simulink model "gtm_design_lpv"  (R2021b)
settings: Solver=VariableStepAuto  StartTime=0.0  StopTime=10  FixedStep=0.005  MaxStep=0.005  RelTol=1e-3
StopFcn:
  | MWSout=grabmws(bdroot);
  | MWSout.lastrun=datestr(now);
values from neighbouring files (symbols this model uses):
  s = tf('s')    [SingleDOF.m]    (also in main.m; mainSimple.m; newmain.m)
undefined symbols (not defined in the file or in its folder): Aero, aftfuel, aftfuel_pos, AILL, AILLC, AILR, AILRC, alpha_deg, altitude_ft, Ax_g, Ay_g, Az_g, b, beta_deg, bias, BRAKEC, Cbar, cg_pos0, cg_shift_gear, DamageCase, DamageModels, DamageOnsetTime, Earth, ELLIB, ELLIBC, ELLOB, ELLOBC, ELRIB, ELRIBC, ELROB, ELROBC, engl_ang, engl_pos, engr_ang, engr_pos, FLAPLIB, FLAPLIC, FLAPLOB, FLAPLOC, FLAPRIB, FLAPRIC, FLAPROB, FLAPROC, ft, FuelUsed_Init, fwdfuel, fwdfuel_pos, GEAR, GEARC, Inertia0, Inertia_shift_gear, Ixx_model, Iyy_model, Izz_model, KTAS, LandingGear, LengON, LinearizeModeOn, NAV_altitude_m, NAV_latitude_deg ... (+51)
libraries: simulink_extras x63, simulink_need_slupdate x30, LPVBlockLibrary x20, aerolibconvert2 x6, aerolibtransform2 x5, uavalgslib x4, UserContent_lib x3, simulink x3, robotcorelib x1, uavutilslib x1
(part 5 of 8)

== system gtm_design_lpv/GTM_T2/Sensors/MIDG II 50 Hz ==
  AuxVars : Inport
  EOM_State : Inport  Port=2
  0.01 deg Resolution : Quantizer  QuantizationInterval=0.01
  0.01 deg Resolution1 : Quantizer  QuantizationInterval=0.01
  0.01 deg Resolution2 : Quantizer  QuantizationInterval=0.01
  0.01 m Resolution1 : Quantizer  QuantizationInterval=0.01
  0.01 m/s Resolution : Quantizer  QuantizationInterval=0.01
  0.01 m/s Resolution1 : Quantizer  QuantizationInterval=0.01
  0.01 m/s Resolution2 : Quantizer  QuantizationInterval=0.01
  1e-7 deg Resolution2 : Quantizer  QuantizationInterval=1e-7
  1e-7 deg Resolution3 : Quantizer  QuantizationInterval=1e-7
  Bus Selector3 : BusSelector  OutputSignals=phi,theta,psi,latitude,longitude,altitude
  Bus Selector8 : BusSelector  OutputSignals=Vn,Ve,Vd
  Bus to Vector : BusToVector
  Gain10 : Gain  Gain=0.5144
  Gain11 : Gain  Gain=-0.5144
  Gain12 : Gain  Gain=0.3048
  Gain{13..17} (5 alike) : Gain  Gain=180/pi
  Gain9 : Gain  Gain=0.5144
  MIDG Labels : Subsystem
  MIDG bus : BusCreator  Inputs=9
  Map+/-180 : Subsystem
  Rate Transition : RateTransition
  Scope{,1..4} (5 alike) : Scope
  Selector{,1..3} (4 alike) : Selector  InputPortWidth=9  IndexOptions=Index vector (dialog)  Indices=4  OutputSizes=1
  Sensor Model7 : Subsystem  mask(Sensor Model){noise_on=SensorNoise.On, sigma=SensorNoise.MIDG.psi.Std, seed=878232, bias=SensorNoise.MIDG.psi.Bias, scf=SensorNoise.MIDG.psi.Scf}
      mask prompts: noise_on "on/off"; scf "scale factor:"
      mask help:
      | Add bias, scale factor, and white noise to a signal
      |
      | - 'on/off': 1 = noise on, 0 = noise off.
      | - 'sigma' : Standard deviation of white noise.
      | - 'seed'  : Random number seed. Generated numbers
      |   change between each simulation run, but the random number
      |   sequences do not change between Matlab sessions unless a
      |   new seed is specified.
      | - 'bias'  : Constant mean value offset of white noise.
      | - 'scale factor' : Scale factor applied to original signal.
      mask Display: disp('bias/scf/noise')
  Sensor Model8 : Subsystem  mask(Sensor Model){noise_on=SensorNoise.On, sigma=SensorNoise.MIDG.theta.Std, seed=878231, bias=SensorNoise.MIDG.theta.Bias, scf=SensorNoise.MIDG.theta.Scf}
      mask prompts: noise_on "on/off"; scf "scale factor:"
      mask help:
      | Add bias, scale factor, and white noise to a signal
      |
      | - 'on/off': 1 = noise on, 0 = noise off.
      | - 'sigma' : Standard deviation of white noise.
      | - 'seed'  : Random number seed. Generated numbers
      |   change between each simulation run, but the random number
      |   sequences do not change between Matlab sessions unless a
      |   new seed is specified.
      | - 'bias'  : Constant mean value offset of white noise.
      | - 'scale factor' : Scale factor applied to original signal.
      mask Display: disp('bias/scf/noise')
  Sensor Model9 : Subsystem  mask(Sensor Model){noise_on=SensorNoise.On, sigma=SensorNoise.MIDG.phi.Std, seed=878230, bias=SensorNoise.MIDG.phi.Bias, scf=SensorNoise.MIDG.phi.Scf}
      mask prompts: noise_on "on/off"; scf "scale factor:"
      mask help:
      | Add bias, scale factor, and white noise to a signal
      |
      | - 'on/off': 1 = noise on, 0 = noise off.
      | - 'sigma' : Standard deviation of white noise.
      | - 'seed'  : Random number seed. Generated numbers
      |   change between each simulation run, but the random number
      |   sequences do not change between Matlab sessions unless a
      |   new seed is specified.
      | - 'bias'  : Constant mean value offset of white noise.
      | - 'scale factor' : Scale factor applied to original signal.
      mask Display: disp('bias/scf/noise')
  TimeDelay with IC feedthrough : Subsystem  mask{TimeDelay=40e-3}
      mask prompts: TimeDelay "Time Delay (sec)"
      mask help:
      | Implements Continuous Time Transport Delay with initial
      | outputs set to feedthrough with no delay.
      |
      |   output = input;   for t<TimeDelay
      |   output = input(t-tdelay); for t>=TimeDelay
  Zero-Order Hold : ZeroOrderHold  SampleTime=round(1/Timestep/50)*Timestep
  MIDG : Outport
  wires:
  Bus to Vector/1 -> Selector/1, TimeDelay with IC feedthrough/1(I)
  TimeDelay with IC feedthrough/1(O) -> Selector1/1, Zero-Order Hold/1
  MIDG bus/1 -> Bus to Vector/1
  Zero-Order Hold/1 -> Selector2/1, Rate Transition/1
  EOM_State/1 -> Bus Selector3/1
  Bus Selector3/1 -> Gain13/1  "<phi>"
  Bus Selector3/2 -> Gain14/1  "<theta>"
  Bus Selector3/3 -> Gain15/1  "<psi>"
  Sensor Model7/1(Out1) -> 0.01 deg Resolution2/1
  Sensor Model8/1(Out1) -> 0.01 deg Resolution1/1
  Sensor Model9/1(Out1) -> 0.01 deg Resolution/1
  0.01 deg Resolution/1 -> MIDG bus/1  "phi"
  0.01 deg Resolution1/1 -> MIDG bus/2  "theta"
  0.01 deg Resolution2/1 -> Map+/-180/1(I)  "psi"
  1e-7 deg Resolution2/1 -> Scope/1, MIDG bus/4  "latitude"
  1e-7 deg Resolution3/1 -> MIDG bus/5  "longitude"
  0.01 m Resolution1/1 -> MIDG bus/6  "altitude"
  Gain9/1 -> 0.01 m/s Resolution/1
  Gain10/1 -> 0.01 m/s Resolution1/1
  Gain11/1 -> 0.01 m/s Resolution2/1
  Gain12/1 -> 0.01 m Resolution1/1
  0.01 m/s Resolution/1 -> MIDG bus/7  "Vn"
  0.01 m/s Resolution1/1 -> MIDG bus/8  "Ve"
  Gain13/1 -> Sensor Model9/1(In1)
  Gain14/1 -> Sensor Model8/1(In1)
  Gain15/1 -> Sensor Model7/1(In1)
  Gain16/1 -> 1e-7 deg Resolution2/1
  Gain17/1 -> 1e-7 deg Resolution3/1
  Bus Selector8/1 -> Gain9/1  "<Vn>"
  Bus Selector8/2 -> Gain10/1  "<Ve>"
  Bus Selector8/3 -> Gain11/1  "<Vd>"
  Bus Selector3/4 -> Gain16/1  "<latitude>"
  Bus Selector3/5 -> Gain17/1  "<longitude>"
  Bus Selector3/6 -> Gain12/1  "<altitude>"
  AuxVars/1 -> Bus Selector8/1
  Map+/-180/1(O) -> MIDG bus/3  "psi"
  MIDG Labels/1(O) -> MIDG/1
  0.01 m/s Resolution2/1 -> MIDG bus/9  "Vu"
  Rate Transition/1 -> Selector3/1, MIDG Labels/1(I)
  Selector/1 -> Scope1/1
  Selector1/1 -> Scope2/1
  Selector2/1 -> Scope3/1
  Selector3/1 -> Scope4/1

== system gtm_design_lpv/GTM_T2/Sensors/Surface Pots ==
  SurfacePos : Inport
  Bus Selector : BusSelector  OutputSignals=ELLOB,ELLIB,ELROB,ELRIB,AILL,AILR,RUDU,RUDL,FLAPLIB,FLAPLOB,FLAPRIB,FLAPROB  OutputAsBus=on
  Sensor Model5 : Subsystem  mask(Sensor Model){noise_on=SensorNoise.On, sigma=SensorNoise.pots.Std, seed=878239, bias=SensorNoise.pots.Bias, scf=SensorNoise.pots.Scf}
      mask prompts: noise_on "on/off"; scf "scale factor:"
      mask help:
      | Add bias, scale factor, and white noise to a signal
      |
      | - 'on/off': 1 = noise on, 0 = noise off.
      | - 'sigma' : Standard deviation of white noise.
      | - 'seed'  : Random number seed. Generated numbers
      |   change between each simulation run, but the random number
      |   sequences do not change between Matlab sessions unless a
      |   new seed is specified.
      | - 'bias'  : Constant mean value offset of white noise.
      | - 'scale factor' : Scale factor applied to original signal.
      mask Display: disp('bias/scf/noise')
  Surface Labels : Subsystem
  Pots : Outport
  wires:
  Bus Selector/1 -> Sensor Model5/1(In1)
  SurfacePos/1 -> Bus Selector/1
  Sensor Model5/1(Out1) -> Surface Labels/1(I)
  Surface Labels/1(O) -> Pots/1

== system gtm_design_lpv/GTM_T2/TransportDelay/AntiAliasing ==
  I : Inport
  Bus Assignment : BusAssignment  AssignedSignals=AirData.alpha_deg,AirData.beta_deg,AirData.qbar_psf,AirData.KTAS,AirData.TEMPAMB_degF,AirData.altitude_ft,MAG3.p_deg,MAG3.q_deg,MAG3.r_deg,MAG3.Ax_g,MAG3.Ay_g,MAG3.Az_g,SurfacePos.ELLOB,SurfacePos.ELLIB,SurfacePos.ELROB,SurfacePos.ELRIB,SurfacePos.AILL,SurfacePos.AILR,SurfacePos.RUDU,SurfacePos.RUDL,SurfacePos.FLAPLIB,SurfacePos.FLAPLOB,SurfacePos.FLAPRIB,SurfacePos.FLAPROB
  Bus Selector : BusSelector  OutputSignals=AirData.alpha_deg,AirData.beta_deg,AirData.qbar_psf,AirData.KTAS,AirData.TEMPAMB_degF,AirData.altitude_ft,MAG3.p_deg,MAG3.q_deg,MAG3.r_deg,MAG3.Ax_g,MAG3.Ay_g,MAG3.Az_g,SurfacePos.ELLOB,SurfacePos.ELLIB,SurfacePos.ELROB,SurfacePos.ELRIB,SurfacePos.AILL,SurfacePos.AILR,SurfacePos.RUDU,SurfacePos.RUDL,SurfacePos.FLAPLIB,SurfacePos.FLAPLOB,SurfacePos.FLAPRIB,SurfacePos.FLAPROB  OutputAsBus=on
  Bus to Vector : BusToVector
  Demux : Demux  Outputs=24
  First Order Filter Continuous : Subsystem  mask(first order filter){tau=1/2/pi/16}
      mask help:
      | __1__
      |  tau s+1
      |
      | First order filter  transfer function
      | with integrator IC = input  at time=0
      |
      | Uses continuous time integrator.
      mask Display: fprintf('  1\n--------------\n %2.1g s + 1', tau)
  O : Outport
  wires:
  Bus to Vector/1 -> First Order Filter Continuous/1(In)
  I/1 -> Bus Selector/1, Bus Assignment/1
  Bus Selector/1 -> Bus to Vector/1
  First Order Filter Continuous/1(Out) -> Demux/1
  Bus Assignment/1 -> O/1
  Demux/1 -> Bus Assignment/2
  Demux/2 -> Bus Assignment/3
  Demux/3 -> Bus Assignment/4
  Demux/4 -> Bus Assignment/5
  Demux/5 -> Bus Assignment/6
  Demux/6 -> Bus Assignment/7
  Demux/7 -> Bus Assignment/8
  Demux/8 -> Bus Assignment/9
  Demux/9 -> Bus Assignment/10
  Demux/10 -> Bus Assignment/11
  Demux/11 -> Bus Assignment/12
  Demux/12 -> Bus Assignment/13
  Demux/13 -> Bus Assignment/14
  Demux/14 -> Bus Assignment/15
  Demux/15 -> Bus Assignment/16
  Demux/16 -> Bus Assignment/17
  Demux/17 -> Bus Assignment/18
  Demux/18 -> Bus Assignment/19
  Demux/19 -> Bus Assignment/20
  Demux/20 -> Bus Assignment/21
  Demux/21 -> Bus Assignment/22
  Demux/22 -> Bus Assignment/23
  Demux/23 -> Bus Assignment/24
  Demux/24 -> Bus Assignment/25

== system gtm_design_lpv/GTM_T2/TransportDelay/Transport Delay on Bus ==
  In : Inport
  Bus Creator : BusCreator  Inputs=5
  Bus Selector : BusSelector  OutputSignals=AirData,MIDG,MAG3,SurfacePos,Engines
  BusDelay : Subsystem
  BusDelay1 : Subsystem
  BusDelay2 : Subsystem
  BusDelay3 : Subsystem
  BusDelay4 : Subsystem
  Out : Outport
  wires:
  In/1 -> Bus Selector/1
  Bus Selector/1 -> BusDelay/1(In1)  "<AirData>"
  Bus Selector/2 -> BusDelay1/1(In1)  "<MIDG>"
  Bus Selector/3 -> BusDelay2/1(In1)  "<MAG3>"
  Bus Selector/4 -> BusDelay3/1(In1)  "<SurfacePos>"
  Bus Selector/5 -> BusDelay4/1(In1)  "<Engines>"
  BusDelay/1(Out1) -> Bus Creator/1  "AirData"
  BusDelay1/1(Out1) -> Bus Creator/2  "MIDG"
  BusDelay2/1(Out1) -> Bus Creator/3  "MAG3"
  BusDelay3/1(Out1) -> Bus Creator/4  "SurfacePos"
  BusDelay4/1(Out1) -> Bus Creator/5  "Engines"
  Bus Creator/1 -> Out/1

== system gtm_design_lpv/GTM_T2/TransportDelay/Transport Delay on Bus1 ==
  In : Inport
  BusDelay : Subsystem
  Out : Outport
  wires:
  In/1 -> BusDelay/1(In1)
  BusDelay/1(Out1) -> Out/1

== system gtm_design_lpv/Navigation and Guidance/Orbit Following/Map 0_360 ==
  I : Inport
  Constant : Constant  Value=2*pi
  Constant1 : Constant  Value=0
  Gain : Gain  Gain=180/pi
  Sum : Sum  Inputs=|++
  ifnegadd2pi : Switch
  O : Outport
  wires:
  Gain/1 -> O/1
  Constant1/1 -> ifnegadd2pi/1
  Constant/1 -> ifnegadd2pi/3
  ifnegadd2pi/1 -> Sum/2
  Sum/1 -> Gain/1
  I/1 -> ifnegadd2pi/2, Sum/1

== system gtm_design_lpv/Navigation and Guidance/Orbit Following/VecNorm ==
  I : Inport
  Math Function2 : Math  Operator=sqrt  SignedPower=on  SaturateOnIntegerOverflow=on
  Product : Product  RndMeth=Zero
  Sum of Elements : Sum  Inputs=+
  O : Outport
  wires:
  Math Function2/1 -> O/1
  I/1 -> Product/1, Product/2
  Product/1 -> Sum of Elements/1
  Sum of Elements/1 -> Math Function2/1

== system gtm_design_lpv/Navigation and Guidance/Waypoint Following/Map 0_360 ==
  I : Inport
  Constant : Constant  Value=2*pi
  Constant1 : Constant  Value=0
  Gain : Gain  Gain=180/pi
  Sum : Sum  Inputs=|++
  ifnegadd2pi : Switch
  O : Outport
  wires:
  Gain/1 -> O/1
  Constant1/1 -> ifnegadd2pi/1
  Constant/1 -> ifnegadd2pi/3
  ifnegadd2pi/1 -> Sum/2
  Sum/1 -> Gain/1
  I/1 -> ifnegadd2pi/2, Sum/1

== system gtm_design_lpv/Navigation and Guidance/Waypoint Following/VecNorm ==
  I : Inport
  Math Function2 : Math  Operator=sqrt  SignedPower=on  SaturateOnIntegerOverflow=on
  Product : Product  RndMeth=Zero
  Sum of Elements : Sum  Inputs=+
  O : Outport
  wires:
  Math Function2/1 -> O/1
  I/1 -> Product/1, Product/2
  Product/1 -> Sum of Elements/1
  Sum of Elements/1 -> Math Function2/1

== system gtm_design_lpv/Navigation and Guidance1/Orbit Following/Map 0_360 ==
  I : Inport
  Constant : Constant  Value=2*pi
  Constant1 : Constant  Value=0
  Gain : Gain  Gain=180/pi
  Sum : Sum  Inputs=|++
  ifnegadd2pi : Switch
  O : Outport
  wires:
  Gain/1 -> O/1
  Constant1/1 -> ifnegadd2pi/1
  Constant/1 -> ifnegadd2pi/3
  ifnegadd2pi/1 -> Sum/2
  Sum/1 -> Gain/1
  I/1 -> ifnegadd2pi/2, Sum/1

== system gtm_design_lpv/Navigation and Guidance1/Orbit Following/VecNorm ==
  I : Inport
  Math Function2 : Math  Operator=sqrt  SignedPower=on  SaturateOnIntegerOverflow=on
  Product : Product  RndMeth=Zero
  Sum of Elements : Sum  Inputs=+
  O : Outport
  wires:
  Math Function2/1 -> O/1
  I/1 -> Product/1, Product/2
  Product/1 -> Sum of Elements/1
  Sum of Elements/1 -> Math Function2/1

== system gtm_design_lpv/Navigation and Guidance1/Waypoint Following/Map 0_360 ==
  I : Inport
  Constant : Constant  Value=2*pi
  Constant1 : Constant  Value=0
  Gain : Gain  Gain=180/pi
  Sum : Sum  Inputs=|++
  ifnegadd2pi : Switch
  O : Outport
  wires:
  Gain/1 -> O/1
  Constant1/1 -> ifnegadd2pi/1
  Constant/1 -> ifnegadd2pi/3
  ifnegadd2pi/1 -> Sum/2
  Sum/1 -> Gain/1
  I/1 -> ifnegadd2pi/2, Sum/1

== system gtm_design_lpv/Navigation and Guidance1/Waypoint Following/VecNorm ==
  I : Inport
  Math Function2 : Math  Operator=sqrt  SignedPower=on  SaturateOnIntegerOverflow=on
  Product : Product  RndMeth=Zero
  Sum of Elements : Sum  Inputs=+
  O : Outport
  wires:
  Math Function2/1 -> O/1
  I/1 -> Product/1, Product/2
  Product/1 -> Sum of Elements/1
  Sum of Elements/1 -> Math Function2/1

== system gtm_design_lpv/GTM_T2/A//C parameters/Inertia//Mass//CG Shift/DamageEffects ==
  In : Inport
  Gain1 : Constant  Value=dInertiaDamage
  Squeeze2 : Squeeze
  Value(ndx,:) : Selector  NumberOfDimensions=2  IndexMode=Zero-based  InputPortWidth=3  IndexOptions=Index vector (port),Select all  Indices=[1 3],1  OutputSizes=1,1
  dInertia : Outport
  wires:
  Squeeze2/1 -> dInertia/1
  Value(ndx,:)/1 -> Squeeze2/1
  Gain1/1 -> Value(ndx,:)/1
  In/1 -> Value(ndx,:)/2

== system gtm_design_lpv/GTM_T2/A//C parameters/Inertia//Mass//CG Shift/FuelBurnEffects ==
  In : Inport
  Mux : Mux
  Polyval : Subsystem  mask{p=Ixx_model}
      mask prompts: p "Polynomial"
      mask help:
      | Embedded MATLAB version of the polyval block.
      | Input polynomial coefficients as a vector in descending order.
      mask Display:
      | disp('y = P(u)\n')
      | disp(['\nO(P) = ' num2str(length(p)-1)])
  Polyval1 : Subsystem  mask{p=Iyy_model}
      mask prompts: p "Polynomial"
      mask help:
      | Embedded MATLAB version of the polyval block.
      | Input polynomial coefficients as a vector in descending order.
      mask Display:
      | disp('y = P(u)\n')
      | disp(['\nO(P) = ' num2str(length(p)-1)])
  Polyval2 : Subsystem  mask{p=Izz_model}
      mask prompts: p "Polynomial"
      mask help:
      | Embedded MATLAB version of the polyval block.
      | Input polynomial coefficients as a vector in descending order.
      mask Display:
      | disp('y = P(u)\n')
      | disp(['\nO(P) = ' num2str(length(p)-1)])
  xCG6 : Constant  Value=zeros(1,3)
  dInertia : Outport
  wires:
  Mux/1 -> dInertia/1
  Polyval2/1(Out1) -> Mux/3
  Polyval1/1(Out1) -> Mux/2
  Polyval/1(Out1) -> Mux/1
  xCG6/1 -> Mux/4
  In/1 -> Polyval2/1(In1), Polyval1/1(In1), Polyval/1(In1)

== system gtm_design_lpv/GTM_T2/A//C parameters/Inertia//Mass//CG Shift/cg//weight ==
  DamageCase : Inport
  Gain1 : Constant  Value=dMassDamage
  Gain2 : Constant  Value=dCGDamage
  Squeeze1 : Squeeze
  Squeeze2 : Squeeze
  Value(ndx,:) : Selector  IndexMode=Zero-based  IndexOptions=Index vector (port)  Indices=[1 3]  OutputSizes=1
  Value(ndx,:)1 : Selector  NumberOfDimensions=2  IndexMode=Zero-based  InputPortWidth=3  IndexOptions=Index vector (port),Select all  Indices=[1 3],1  OutputSizes=1,1
  dCG : Outport
  dweight : Outport  Port=2
  wires:
  Squeeze2/1 -> dweight/1
  Squeeze1/1 -> dCG/1
  Value(ndx,:)/1 -> Squeeze2/1
  Gain1/1 -> Value(ndx,:)/1
  DamageCase/1 -> Value(ndx,:)1/2, Value(ndx,:)/2
  Value(ndx,:)1/1 -> Squeeze1/1
  Gain2/1 -> Value(ndx,:)1/1

== system gtm_design_lpv/GTM_T2/Actuators/Acutator Dynamics/ElevatorLIBServo ==
  In : Inport
  Constant : Constant  Value=Bias
  Gain : Gain  Gain=2*pi*freq  SaturateOnIntegerOverflow=on  OutDataTypeStr=Inherit: Same as input  ParamDataTypeStr=Inherit: Same as input
  Integrator : Integrator  InitialConditionSource=external  LimitOutput=on  UpperSaturationLimit=POS_hi  LowerSaturationLimit=POS_lo  IgnoreLimit=on
  Rate Limiter : Saturate  UpperLimit=RL  LowerLimit=-RL
  Sum : Sum  Inputs=-+|  InputSameDT=on  SaturateOnIntegerOverflow=on  OutDataTypeStr=Inherit: Same as first input
  Sum1 : Sum  Inputs=++|  InputSameDT=on  SaturateOnIntegerOverflow=on  OutDataTypeStr=Inherit: Same as first input
  Out : Outport  PortDimensions=1
  wires:
  Constant/1 -> Sum1/1
  Sum1/1 -> Integrator/2, Sum/2
  In/1 -> Sum1/2
  Rate Limiter/1 -> Integrator/1  "Ydot_lim"
  Integrator/1 -> Out/1, Sum/1  "Y"
  Sum/1 -> Gain/1  "Error"
  Gain/1 -> Rate Limiter/1  "Ydot"

== system gtm_design_lpv/GTM_T2/Actuators/Acutator Dynamics/ElevatorLOBServo ==
  In : Inport
  Constant : Constant  Value=Bias
  Gain : Gain  Gain=2*pi*freq  SaturateOnIntegerOverflow=on  OutDataTypeStr=Inherit: Same as input  ParamDataTypeStr=Inherit: Same as input
  Integrator : Integrator  InitialConditionSource=external  LimitOutput=on  UpperSaturationLimit=POS_hi  LowerSaturationLimit=POS_lo  IgnoreLimit=on
  Rate Limiter : Saturate  UpperLimit=RL  LowerLimit=-RL
  Sum : Sum  Inputs=-+|  InputSameDT=on  SaturateOnIntegerOverflow=on  OutDataTypeStr=Inherit: Same as first input
  Sum1 : Sum  Inputs=++|  InputSameDT=on  SaturateOnIntegerOverflow=on  OutDataTypeStr=Inherit: Same as first input
  Out : Outport  PortDimensions=1
  wires:
  Constant/1 -> Sum1/1
  Sum1/1 -> Integrator/2, Sum/2
  In/1 -> Sum1/2
  Rate Limiter/1 -> Integrator/1  "Ydot_lim"
  Integrator/1 -> Out/1, Sum/1  "Y"
  Sum/1 -> Gain/1  "Error"
  Gain/1 -> Rate Limiter/1  "Ydot"

== system gtm_design_lpv/GTM_T2/Actuators/Acutator Dynamics/ElevatorRIBServo ==
  In : Inport
  Constant : Constant  Value=Bias
  Gain : Gain  Gain=2*pi*freq  SaturateOnIntegerOverflow=on  OutDataTypeStr=Inherit: Same as input  ParamDataTypeStr=Inherit: Same as input
  Integrator : Integrator  InitialConditionSource=external  LimitOutput=on  UpperSaturationLimit=POS_hi  LowerSaturationLimit=POS_lo  IgnoreLimit=on
  Rate Limiter : Saturate  UpperLimit=RL  LowerLimit=-RL
  Sum : Sum  Inputs=-+|  InputSameDT=on  SaturateOnIntegerOverflow=on  OutDataTypeStr=Inherit: Same as first input
  Sum1 : Sum  Inputs=++|  InputSameDT=on  SaturateOnIntegerOverflow=on  OutDataTypeStr=Inherit: Same as first input
  Out : Outport  PortDimensions=1
  wires:
  Constant/1 -> Sum1/1
  Sum1/1 -> Integrator/2, Sum/2
  In/1 -> Sum1/2
  Rate Limiter/1 -> Integrator/1  "Ydot_lim"
  Integrator/1 -> Out/1, Sum/1  "Y"
  Sum/1 -> Gain/1  "Error"
  Gain/1 -> Rate Limiter/1  "Ydot"

== system gtm_design_lpv/GTM_T2/Actuators/Acutator Dynamics/ElevatorROBServo ==
  In : Inport
  Constant : Constant  Value=Bias
  Gain : Gain  Gain=2*pi*freq  SaturateOnIntegerOverflow=on  OutDataTypeStr=Inherit: Same as input  ParamDataTypeStr=Inherit: Same as input
  Integrator : Integrator  InitialConditionSource=external  LimitOutput=on  UpperSaturationLimit=POS_hi  LowerSaturationLimit=POS_lo  IgnoreLimit=on
  Rate Limiter : Saturate  UpperLimit=RL  LowerLimit=-RL
  Sum : Sum  Inputs=-+|  InputSameDT=on  SaturateOnIntegerOverflow=on  OutDataTypeStr=Inherit: Same as first input
  Sum1 : Sum  Inputs=++|  InputSameDT=on  SaturateOnIntegerOverflow=on  OutDataTypeStr=Inherit: Same as first input
  Out : Outport  PortDimensions=1
  wires:
  Constant/1 -> Sum1/1
  Sum1/1 -> Integrator/2, Sum/2
  In/1 -> Sum1/2
  Rate Limiter/1 -> Integrator/1  "Ydot_lim"
  Integrator/1 -> Out/1, Sum/1  "Y"
  Sum/1 -> Gain/1  "Error"
  Gain/1 -> Rate Limiter/1  "Ydot"

== system gtm_design_lpv/GTM_T2/Actuators/Acutator Dynamics/FlapLIBServo ==
  In : Inport
  Constant : Constant  Value=Bias
  Gain : Gain  Gain=2*pi*freq  SaturateOnIntegerOverflow=on  OutDataTypeStr=Inherit: Same as input  ParamDataTypeStr=Inherit: Same as input
  Integrator : Integrator  InitialConditionSource=external  LimitOutput=on  UpperSaturationLimit=POS_hi  LowerSaturationLimit=POS_lo  IgnoreLimit=on
  Rate Limiter : Saturate  UpperLimit=RL  LowerLimit=-RL
  Sum : Sum  Inputs=-+|  InputSameDT=on  SaturateOnIntegerOverflow=on  OutDataTypeStr=Inherit: Same as first input
  Sum1 : Sum  Inputs=++|  InputSameDT=on  SaturateOnIntegerOverflow=on  OutDataTypeStr=Inherit: Same as first input
  Out : Outport  PortDimensions=1
  wires:
  Constant/1 -> Sum1/1
  Sum1/1 -> Integrator/2, Sum/2
  In/1 -> Sum1/2
  Rate Limiter/1 -> Integrator/1  "Ydot_lim"
  Integrator/1 -> Out/1, Sum/1  "Y"
  Sum/1 -> Gain/1  "Error"
  Gain/1 -> Rate Limiter/1  "Ydot"

== system gtm_design_lpv/GTM_T2/Actuators/Acutator Dynamics/FlapLOBServo ==
  In : Inport
  Constant : Constant  Value=Bias
  Gain : Gain  Gain=2*pi*freq  SaturateOnIntegerOverflow=on  OutDataTypeStr=Inherit: Same as input  ParamDataTypeStr=Inherit: Same as input
  Integrator : Integrator  InitialConditionSource=external  LimitOutput=on  UpperSaturationLimit=POS_hi  LowerSaturationLimit=POS_lo  IgnoreLimit=on
  Rate Limiter : Saturate  UpperLimit=RL  LowerLimit=-RL
  Sum : Sum  Inputs=-+|  InputSameDT=on  SaturateOnIntegerOverflow=on  OutDataTypeStr=Inherit: Same as first input
  Sum1 : Sum  Inputs=++|  InputSameDT=on  SaturateOnIntegerOverflow=on  OutDataTypeStr=Inherit: Same as first input
  Out : Outport  PortDimensions=1
  wires:
  Constant/1 -> Sum1/1
  Sum1/1 -> Integrator/2, Sum/2
  In/1 -> Sum1/2
  Rate Limiter/1 -> Integrator/1  "Ydot_lim"
  Integrator/1 -> Out/1, Sum/1  "Y"
  Sum/1 -> Gain/1  "Error"
  Gain/1 -> Rate Limiter/1  "Ydot"

== system gtm_design_lpv/GTM_T2/Actuators/Acutator Dynamics/FlapRIBServo ==
  In : Inport
  Constant : Constant  Value=Bias
  Gain : Gain  Gain=2*pi*freq  SaturateOnIntegerOverflow=on  OutDataTypeStr=Inherit: Same as input  ParamDataTypeStr=Inherit: Same as input
  Integrator : Integrator  InitialConditionSource=external  LimitOutput=on  UpperSaturationLimit=POS_hi  LowerSaturationLimit=POS_lo  IgnoreLimit=on
  Rate Limiter : Saturate  UpperLimit=RL  LowerLimit=-RL
  Sum : Sum  Inputs=-+|  InputSameDT=on  SaturateOnIntegerOverflow=on  OutDataTypeStr=Inherit: Same as first input
  Sum1 : Sum  Inputs=++|  InputSameDT=on  SaturateOnIntegerOverflow=on  OutDataTypeStr=Inherit: Same as first input
  Out : Outport  PortDimensions=1
  wires:
  Constant/1 -> Sum1/1
  Sum1/1 -> Integrator/2, Sum/2
  In/1 -> Sum1/2
  Rate Limiter/1 -> Integrator/1  "Ydot_lim"
  Integrator/1 -> Out/1, Sum/1  "Y"
  Sum/1 -> Gain/1  "Error"
  Gain/1 -> Rate Limiter/1  "Ydot"

== system gtm_design_lpv/GTM_T2/Actuators/Acutator Dynamics/FlapROBServo ==
  In : Inport
  Constant : Constant  Value=Bias
  Gain : Gain  Gain=2*pi*freq  SaturateOnIntegerOverflow=on  OutDataTypeStr=Inherit: Same as input  ParamDataTypeStr=Inherit: Same as input
  Integrator : Integrator  InitialConditionSource=external  LimitOutput=on  UpperSaturationLimit=POS_hi  LowerSaturationLimit=POS_lo  IgnoreLimit=on
  Rate Limiter : Saturate  UpperLimit=RL  LowerLimit=-RL
  Sum : Sum  Inputs=-+|  InputSameDT=on  SaturateOnIntegerOverflow=on  OutDataTypeStr=Inherit: Same as first input
  Sum1 : Sum  Inputs=++|  InputSameDT=on  SaturateOnIntegerOverflow=on  OutDataTypeStr=Inherit: Same as first input
  Out : Outport  PortDimensions=1
  wires:
  Constant/1 -> Sum1/1
  Sum1/1 -> Integrator/2, Sum/2
  In/1 -> Sum1/2
  Rate Limiter/1 -> Integrator/1  "Ydot_lim"
  Integrator/1 -> Out/1, Sum/1  "Y"
  Sum/1 -> Gain/1  "Error"
  Gain/1 -> Rate Limiter/1  "Ydot"

== system gtm_design_lpv/GTM_T2/Actuators/Acutator Dynamics/LeftAileronServo ==
  In : Inport
  Constant : Constant  Value=Bias
  Gain : Gain  Gain=2*pi*freq  SaturateOnIntegerOverflow=on  OutDataTypeStr=Inherit: Same as input  ParamDataTypeStr=Inherit: Same as input
  Integrator : Integrator  InitialConditionSource=external  LimitOutput=on  UpperSaturationLimit=POS_hi  LowerSaturationLimit=POS_lo  IgnoreLimit=on
  Rate Limiter : Saturate  UpperLimit=RL  LowerLimit=-RL
  Sum : Sum  Inputs=-+|  InputSameDT=on  SaturateOnIntegerOverflow=on  OutDataTypeStr=Inherit: Same as first input
  Sum1 : Sum  Inputs=++|  InputSameDT=on  SaturateOnIntegerOverflow=on  OutDataTypeStr=Inherit: Same as first input
  Out : Outport  PortDimensions=1
  wires:
  Constant/1 -> Sum1/1
  Sum1/1 -> Integrator/2, Sum/2
  In/1 -> Sum1/2
  Rate Limiter/1 -> Integrator/1  "Ydot_lim"
  Integrator/1 -> Out/1, Sum/1  "Y"
  Sum/1 -> Gain/1  "Error"
  Gain/1 -> Rate Limiter/1  "Ydot"

== system gtm_design_lpv/GTM_T2/Actuators/Acutator Dynamics/LeftIBSpoilerServo ==
  In : Inport
  Constant : Constant  Value=Bias
  Gain : Gain  Gain=2*pi*freq  SaturateOnIntegerOverflow=on  OutDataTypeStr=Inherit: Same as input  ParamDataTypeStr=Inherit: Same as input
  Integrator : Integrator  InitialConditionSource=external  LimitOutput=on  UpperSaturationLimit=POS_hi  LowerSaturationLimit=POS_lo  IgnoreLimit=on
  Rate Limiter : Saturate  UpperLimit=RL  LowerLimit=-RL
  Sum : Sum  Inputs=-+|  InputSameDT=on  SaturateOnIntegerOverflow=on  OutDataTypeStr=Inherit: Same as first input
  Sum1 : Sum  Inputs=++|  InputSameDT=on  SaturateOnIntegerOverflow=on  OutDataTypeStr=Inherit: Same as first input
  Out : Outport  PortDimensions=1
  wires:
  Constant/1 -> Sum1/1
  Sum1/1 -> Integrator/2, Sum/2
  In/1 -> Sum1/2
  Rate Limiter/1 -> Integrator/1  "Ydot_lim"
  Integrator/1 -> Out/1, Sum/1  "Y"
  Sum/1 -> Gain/1  "Error"
  Gain/1 -> Rate Limiter/1  "Ydot"

== system gtm_design_lpv/GTM_T2/Actuators/Acutator Dynamics/LeftOBSpoilerServo ==
  In : Inport
  Constant : Constant  Value=Bias
  Gain : Gain  Gain=2*pi*freq  SaturateOnIntegerOverflow=on  OutDataTypeStr=Inherit: Same as input  ParamDataTypeStr=Inherit: Same as input
  Integrator : Integrator  InitialConditionSource=external  LimitOutput=on  UpperSaturationLimit=POS_hi  LowerSaturationLimit=POS_lo  IgnoreLimit=on
  Rate Limiter : Saturate  UpperLimit=RL  LowerLimit=-RL
  Sum : Sum  Inputs=-+|  InputSameDT=on  SaturateOnIntegerOverflow=on  OutDataTypeStr=Inherit: Same as first input
  Sum1 : Sum  Inputs=++|  InputSameDT=on  SaturateOnIntegerOverflow=on  OutDataTypeStr=Inherit: Same as first input
  Out : Outport  PortDimensions=1
  wires:
  Constant/1 -> Sum1/1
  Sum1/1 -> Integrator/2, Sum/2
  In/1 -> Sum1/2
  Rate Limiter/1 -> Integrator/1  "Ydot_lim"
  Integrator/1 -> Out/1, Sum/1  "Y"
  Sum/1 -> Gain/1  "Error"
  Gain/1 -> Rate Limiter/1  "Ydot"

== system gtm_design_lpv/GTM_T2/Actuators/Acutator Dynamics/RightAileronServo ==
  In : Inport
  Constant : Constant  Value=Bias
  Gain : Gain  Gain=2*pi*freq  SaturateOnIntegerOverflow=on  OutDataTypeStr=Inherit: Same as input  ParamDataTypeStr=Inherit: Same as input
  Integrator : Integrator  InitialConditionSource=external  LimitOutput=on  UpperSaturationLimit=POS_hi  LowerSaturationLimit=POS_lo  IgnoreLimit=on
  Rate Limiter : Saturate  UpperLimit=RL  LowerLimit=-RL
  Sum : Sum  Inputs=-+|  InputSameDT=on  SaturateOnIntegerOverflow=on  OutDataTypeStr=Inherit: Same as first input
  Sum1 : Sum  Inputs=++|  InputSameDT=on  SaturateOnIntegerOverflow=on  OutDataTypeStr=Inherit: Same as first input
  Out : Outport  PortDimensions=1
  wires:
  Constant/1 -> Sum1/1
  Sum1/1 -> Integrator/2, Sum/2
  In/1 -> Sum1/2
  Rate Limiter/1 -> Integrator/1  "Ydot_lim"
  Integrator/1 -> Out/1, Sum/1  "Y"
  Sum/1 -> Gain/1  "Error"
  Gain/1 -> Rate Limiter/1  "Ydot"

== system gtm_design_lpv/GTM_T2/Actuators/Acutator Dynamics/RightIBSpoilerServo ==
  In : Inport
  Constant : Constant  Value=Bias
  Gain : Gain  Gain=2*pi*freq  SaturateOnIntegerOverflow=on  OutDataTypeStr=Inherit: Same as input  ParamDataTypeStr=Inherit: Same as input
  Integrator : Integrator  InitialConditionSource=external  LimitOutput=on  UpperSaturationLimit=POS_hi  LowerSaturationLimit=POS_lo  IgnoreLimit=on
  Rate Limiter : Saturate  UpperLimit=RL  LowerLimit=-RL
  Sum : Sum  Inputs=-+|  InputSameDT=on  SaturateOnIntegerOverflow=on  OutDataTypeStr=Inherit: Same as first input
  Sum1 : Sum  Inputs=++|  InputSameDT=on  SaturateOnIntegerOverflow=on  OutDataTypeStr=Inherit: Same as first input
  Out : Outport  PortDimensions=1
  wires:
  Constant/1 -> Sum1/1
  Sum1/1 -> Integrator/2, Sum/2
  In/1 -> Sum1/2
  Rate Limiter/1 -> Integrator/1  "Ydot_lim"
  Integrator/1 -> Out/1, Sum/1  "Y"
  Sum/1 -> Gain/1  "Error"
  Gain/1 -> Rate Limiter/1  "Ydot"

== system gtm_design_lpv/GTM_T2/Actuators/Acutator Dynamics/RightOBSpoilerServo ==
  In : Inport
  Constant : Constant  Value=Bias
  Gain : Gain  Gain=2*pi*freq  SaturateOnIntegerOverflow=on  OutDataTypeStr=Inherit: Same as input  ParamDataTypeStr=Inherit: Same as input
  Integrator : Integrator  InitialConditionSource=external  LimitOutput=on  UpperSaturationLimit=POS_hi  LowerSaturationLimit=POS_lo  IgnoreLimit=on
  Rate Limiter : Saturate  UpperLimit=RL  LowerLimit=-RL
  Sum : Sum  Inputs=-+|  InputSameDT=on  SaturateOnIntegerOverflow=on  OutDataTypeStr=Inherit: Same as first input
  Sum1 : Sum  Inputs=++|  InputSameDT=on  SaturateOnIntegerOverflow=on  OutDataTypeStr=Inherit: Same as first input
  Out : Outport  PortDimensions=1
  wires:
  Constant/1 -> Sum1/1
  Sum1/1 -> Integrator/2, Sum/2
  In/1 -> Sum1/2
  Rate Limiter/1 -> Integrator/1  "Ydot_lim"
  Integrator/1 -> Out/1, Sum/1  "Y"
  Sum/1 -> Gain/1  "Error"
  Gain/1 -> Rate Limiter/1  "Ydot"

== system gtm_design_lpv/GTM_T2/Actuators/Acutator Dynamics/RudderLServo ==
  In : Inport
  Constant : Constant  Value=Bias
  Gain : Gain  Gain=2*pi*freq  SaturateOnIntegerOverflow=on  OutDataTypeStr=Inherit: Same as input  ParamDataTypeStr=Inherit: Same as input
  Integrator : Integrator  InitialConditionSource=external  LimitOutput=on  UpperSaturationLimit=POS_hi  LowerSaturationLimit=POS_lo  IgnoreLimit=on
  Rate Limiter : Saturate  UpperLimit=RL  LowerLimit=-RL
  Sum : Sum  Inputs=-+|  InputSameDT=on  SaturateOnIntegerOverflow=on  OutDataTypeStr=Inherit: Same as first input
  Sum1 : Sum  Inputs=++|  InputSameDT=on  SaturateOnIntegerOverflow=on  OutDataTypeStr=Inherit: Same as first input
  Out : Outport  PortDimensions=1
  wires:
  Constant/1 -> Sum1/1
  Sum1/1 -> Integrator/2, Sum/2
  In/1 -> Sum1/2
  Rate Limiter/1 -> Integrator/1  "Ydot_lim"
  Integrator/1 -> Out/1, Sum/1  "Y"
  Sum/1 -> Gain/1  "Error"
  Gain/1 -> Rate Limiter/1  "Ydot"

== system gtm_design_lpv/GTM_T2/Actuators/Acutator Dynamics/RudderUServo ==
  In : Inport
  Constant : Constant  Value=Bias
  Gain : Gain  Gain=2*pi*freq  SaturateOnIntegerOverflow=on  OutDataTypeStr=Inherit: Same as input  ParamDataTypeStr=Inherit: Same as input
  Integrator : Integrator  InitialConditionSource=external  LimitOutput=on  UpperSaturationLimit=POS_hi  LowerSaturationLimit=POS_lo  IgnoreLimit=on
  Rate Limiter : Saturate  UpperLimit=RL  LowerLimit=-RL
  Sum : Sum  Inputs=-+|  InputSameDT=on  SaturateOnIntegerOverflow=on  OutDataTypeStr=Inherit: Same as first input
  Sum1 : Sum  Inputs=++|  InputSameDT=on  SaturateOnIntegerOverflow=on  OutDataTypeStr=Inherit: Same as first input
  Out : Outport  PortDimensions=1
  wires:
  Constant/1 -> Sum1/1
  Sum1/1 -> Integrator/2, Sum/2
  In/1 -> Sum1/2
  Rate Limiter/1 -> Integrator/1  "Ydot_lim"
  Integrator/1 -> Out/1, Sum/1  "Y"
  Sum/1 -> Gain/1  "Error"
  Gain/1 -> Rate Limiter/1  "Ydot"

== system gtm_design_lpv/GTM_T2/Actuators/Acutator Dynamics/SteeringServo ==
  In : Inport
  Constant : Constant  Value=Bias
  Gain : Gain  Gain=2*pi*freq  SaturateOnIntegerOverflow=on  OutDataTypeStr=Inherit: Same as input  ParamDataTypeStr=Inherit: Same as input
  Integrator : Integrator  InitialConditionSource=external  LimitOutput=on  UpperSaturationLimit=POS_hi  LowerSaturationLimit=POS_lo  IgnoreLimit=on
  Rate Limiter : Saturate  UpperLimit=RL  LowerLimit=-RL
  Sum : Sum  Inputs=-+|  InputSameDT=on  SaturateOnIntegerOverflow=on  OutDataTypeStr=Inherit: Same as first input
  Sum1 : Sum  Inputs=++|  InputSameDT=on  SaturateOnIntegerOverflow=on  OutDataTypeStr=Inherit: Same as first input
  Out : Outport  PortDimensions=1
  wires:
  Constant/1 -> Sum1/1
  Sum1/1 -> Integrator/2, Sum/2
  In/1 -> Sum1/2
  Rate Limiter/1 -> Integrator/1  "Ydot_lim"
  Integrator/1 -> Out/1, Sum/1  "Y"
  Sum/1 -> Gain/1  "Error"
  Gain/1 -> Rate Limiter/1  "Ydot"

== system gtm_design_lpv/GTM_T2/Actuators/Acutator Dynamics (Unbiased)/ElevatorLIBServo ==
  In : Inport
  Constant : Constant  Value=Bias
  Gain : Gain  Gain=2*pi*freq  SaturateOnIntegerOverflow=on  OutDataTypeStr=Inherit: Same as input  ParamDataTypeStr=Inherit: Same as input
  Integrator : Integrator  InitialConditionSource=external  LimitOutput=on  UpperSaturationLimit=POS_hi  LowerSaturationLimit=POS_lo  IgnoreLimit=on
  Rate Limiter : Saturate  UpperLimit=RL  LowerLimit=-RL
  Sum : Sum  Inputs=-+|  InputSameDT=on  SaturateOnIntegerOverflow=on  OutDataTypeStr=Inherit: Same as first input
  Sum1 : Sum  Inputs=++|  InputSameDT=on  SaturateOnIntegerOverflow=on  OutDataTypeStr=Inherit: Same as first input
  Out : Outport  PortDimensions=1
  wires:
  Gain/1 -> Rate Limiter/1  "Ydot"
  Sum/1 -> Gain/1  "Error"
  Integrator/1 -> Sum/1, Out/1  "Y"
  Rate Limiter/1 -> Integrator/1  "Ydot_lim"
  In/1 -> Sum1/2
  Sum1/1 -> Sum/2, Integrator/2
  Constant/1 -> Sum1/1

== system gtm_design_lpv/GTM_T2/Actuators/Acutator Dynamics (Unbiased)/ElevatorLOBServo ==
  In : Inport
  Constant : Constant  Value=Bias
  Gain : Gain  Gain=2*pi*freq  SaturateOnIntegerOverflow=on  OutDataTypeStr=Inherit: Same as input  ParamDataTypeStr=Inherit: Same as input
  Integrator : Integrator  InitialConditionSource=external  LimitOutput=on  UpperSaturationLimit=POS_hi  LowerSaturationLimit=POS_lo  IgnoreLimit=on
  Rate Limiter : Saturate  UpperLimit=RL  LowerLimit=-RL
  Sum : Sum  Inputs=-+|  InputSameDT=on  SaturateOnIntegerOverflow=on  OutDataTypeStr=Inherit: Same as first input
  Sum1 : Sum  Inputs=++|  InputSameDT=on  SaturateOnIntegerOverflow=on  OutDataTypeStr=Inherit: Same as first input
  Out : Outport  PortDimensions=1
  wires:
  Gain/1 -> Rate Limiter/1  "Ydot"
  Sum/1 -> Gain/1  "Error"
  Integrator/1 -> Sum/1, Out/1  "Y"
  Rate Limiter/1 -> Integrator/1  "Ydot_lim"
  In/1 -> Sum1/2
  Sum1/1 -> Sum/2, Integrator/2
  Constant/1 -> Sum1/1

== system gtm_design_lpv/GTM_T2/Actuators/Acutator Dynamics (Unbiased)/ElevatorRIBServo ==
  In : Inport
  Constant : Constant  Value=Bias
  Gain : Gain  Gain=2*pi*freq  SaturateOnIntegerOverflow=on  OutDataTypeStr=Inherit: Same as input  ParamDataTypeStr=Inherit: Same as input
  Integrator : Integrator  InitialConditionSource=external  LimitOutput=on  UpperSaturationLimit=POS_hi  LowerSaturationLimit=POS_lo  IgnoreLimit=on
  Rate Limiter : Saturate  UpperLimit=RL  LowerLimit=-RL
  Sum : Sum  Inputs=-+|  InputSameDT=on  SaturateOnIntegerOverflow=on  OutDataTypeStr=Inherit: Same as first input
  Sum1 : Sum  Inputs=++|  InputSameDT=on  SaturateOnIntegerOverflow=on  OutDataTypeStr=Inherit: Same as first input
  Out : Outport  PortDimensions=1
  wires:
  Gain/1 -> Rate Limiter/1  "Ydot"
  Sum/1 -> Gain/1  "Error"
  Integrator/1 -> Sum/1, Out/1  "Y"
  Rate Limiter/1 -> Integrator/1  "Ydot_lim"
  In/1 -> Sum1/2
  Sum1/1 -> Sum/2, Integrator/2
  Constant/1 -> Sum1/1

== system gtm_design_lpv/GTM_T2/Actuators/Acutator Dynamics (Unbiased)/ElevatorROBServo ==
  In : Inport
  Constant : Constant  Value=Bias
  Gain : Gain  Gain=2*pi*freq  SaturateOnIntegerOverflow=on  OutDataTypeStr=Inherit: Same as input  ParamDataTypeStr=Inherit: Same as input
  Integrator : Integrator  InitialConditionSource=external  LimitOutput=on  UpperSaturationLimit=POS_hi  LowerSaturationLimit=POS_lo  IgnoreLimit=on
  Rate Limiter : Saturate  UpperLimit=RL  LowerLimit=-RL
  Sum : Sum  Inputs=-+|  InputSameDT=on  SaturateOnIntegerOverflow=on  OutDataTypeStr=Inherit: Same as first input
  Sum1 : Sum  Inputs=++|  InputSameDT=on  SaturateOnIntegerOverflow=on  OutDataTypeStr=Inherit: Same as first input
  Out : Outport  PortDimensions=1
  wires:
  Gain/1 -> Rate Limiter/1  "Ydot"
  Sum/1 -> Gain/1  "Error"
  Integrator/1 -> Sum/1, Out/1  "Y"
  Rate Limiter/1 -> Integrator/1  "Ydot_lim"
  In/1 -> Sum1/2
  Sum1/1 -> Sum/2, Integrator/2
  Constant/1 -> Sum1/1

== system gtm_design_lpv/GTM_T2/Actuators/Acutator Dynamics (Unbiased)/FlapLIBServo ==
  In : Inport
  Constant : Constant  Value=Bias
  Gain : Gain  Gain=2*pi*freq  SaturateOnIntegerOverflow=on  OutDataTypeStr=Inherit: Same as input  ParamDataTypeStr=Inherit: Same as input
  Integrator : Integrator  InitialConditionSource=external  LimitOutput=on  UpperSaturationLimit=POS_hi  LowerSaturationLimit=POS_lo  IgnoreLimit=on
  Rate Limiter : Saturate  UpperLimit=RL  LowerLimit=-RL
  Sum : Sum  Inputs=-+|  InputSameDT=on  SaturateOnIntegerOverflow=on  OutDataTypeStr=Inherit: Same as first input
  Sum1 : Sum  Inputs=++|  InputSameDT=on  SaturateOnIntegerOverflow=on  OutDataTypeStr=Inherit: Same as first input
  Out : Outport  PortDimensions=1
  wires:
  Gain/1 -> Rate Limiter/1  "Ydot"
  Sum/1 -> Gain/1  "Error"
  Integrator/1 -> Sum/1, Out/1  "Y"
  Rate Limiter/1 -> Integrator/1  "Ydot_lim"
  In/1 -> Sum1/2
  Sum1/1 -> Sum/2, Integrator/2
  Constant/1 -> Sum1/1

== system gtm_design_lpv/GTM_T2/Actuators/Acutator Dynamics (Unbiased)/FlapLOBServo ==
  In : Inport
  Constant : Constant  Value=Bias
  Gain : Gain  Gain=2*pi*freq  SaturateOnIntegerOverflow=on  OutDataTypeStr=Inherit: Same as input  ParamDataTypeStr=Inherit: Same as input
  Integrator : Integrator  InitialConditionSource=external  LimitOutput=on  UpperSaturationLimit=POS_hi  LowerSaturationLimit=POS_lo  IgnoreLimit=on
  Rate Limiter : Saturate  UpperLimit=RL  LowerLimit=-RL
  Sum : Sum  Inputs=-+|  InputSameDT=on  SaturateOnIntegerOverflow=on  OutDataTypeStr=Inherit: Same as first input
  Sum1 : Sum  Inputs=++|  InputSameDT=on  SaturateOnIntegerOverflow=on  OutDataTypeStr=Inherit: Same as first input
  Out : Outport  PortDimensions=1
  wires:
  Gain/1 -> Rate Limiter/1  "Ydot"
  Sum/1 -> Gain/1  "Error"
  Integrator/1 -> Sum/1, Out/1  "Y"
  Rate Limiter/1 -> Integrator/1  "Ydot_lim"
  In/1 -> Sum1/2
  Sum1/1 -> Sum/2, Integrator/2
  Constant/1 -> Sum1/1

== system gtm_design_lpv/GTM_T2/Actuators/Acutator Dynamics (Unbiased)/FlapRIBServo ==
  In : Inport
  Constant : Constant  Value=Bias
  Gain : Gain  Gain=2*pi*freq  SaturateOnIntegerOverflow=on  OutDataTypeStr=Inherit: Same as input  ParamDataTypeStr=Inherit: Same as input
  Integrator : Integrator  InitialConditionSource=external  LimitOutput=on  UpperSaturationLimit=POS_hi  LowerSaturationLimit=POS_lo  IgnoreLimit=on
  Rate Limiter : Saturate  UpperLimit=RL  LowerLimit=-RL
  Sum : Sum  Inputs=-+|  InputSameDT=on  SaturateOnIntegerOverflow=on  OutDataTypeStr=Inherit: Same as first input
  Sum1 : Sum  Inputs=++|  InputSameDT=on  SaturateOnIntegerOverflow=on  OutDataTypeStr=Inherit: Same as first input
  Out : Outport  PortDimensions=1
  wires:
  Gain/1 -> Rate Limiter/1  "Ydot"
  Sum/1 -> Gain/1  "Error"
  Integrator/1 -> Sum/1, Out/1  "Y"
  Rate Limiter/1 -> Integrator/1  "Ydot_lim"
  In/1 -> Sum1/2
  Sum1/1 -> Sum/2, Integrator/2
  Constant/1 -> Sum1/1

== system gtm_design_lpv/GTM_T2/Actuators/Acutator Dynamics (Unbiased)/FlapROBServo ==
  In : Inport
  Constant : Constant  Value=Bias
  Gain : Gain  Gain=2*pi*freq  SaturateOnIntegerOverflow=on  OutDataTypeStr=Inherit: Same as input  ParamDataTypeStr=Inherit: Same as input
  Integrator : Integrator  InitialConditionSource=external  LimitOutput=on  UpperSaturationLimit=POS_hi  LowerSaturationLimit=POS_lo  IgnoreLimit=on
  Rate Limiter : Saturate  UpperLimit=RL  LowerLimit=-RL
  Sum : Sum  Inputs=-+|  InputSameDT=on  SaturateOnIntegerOverflow=on  OutDataTypeStr=Inherit: Same as first input
  Sum1 : Sum  Inputs=++|  InputSameDT=on  SaturateOnIntegerOverflow=on  OutDataTypeStr=Inherit: Same as first input
  Out : Outport  PortDimensions=1
  wires:
  Gain/1 -> Rate Limiter/1  "Ydot"
  Sum/1 -> Gain/1  "Error"
  Integrator/1 -> Sum/1, Out/1  "Y"
  Rate Limiter/1 -> Integrator/1  "Ydot_lim"
  In/1 -> Sum1/2
  Sum1/1 -> Sum/2, Integrator/2
  Constant/1 -> Sum1/1

== system gtm_design_lpv/GTM_T2/Actuators/Acutator Dynamics (Unbiased)/LeftAileronServo ==
  In : Inport
  Constant : Constant  Value=Bias
  Gain : Gain  Gain=2*pi*freq  SaturateOnIntegerOverflow=on  OutDataTypeStr=Inherit: Same as input  ParamDataTypeStr=Inherit: Same as input
  Integrator : Integrator  InitialConditionSource=external  LimitOutput=on  UpperSaturationLimit=POS_hi  LowerSaturationLimit=POS_lo  IgnoreLimit=on
  Rate Limiter : Saturate  UpperLimit=RL  LowerLimit=-RL
  Sum : Sum  Inputs=-+|  InputSameDT=on  SaturateOnIntegerOverflow=on  OutDataTypeStr=Inherit: Same as first input
  Sum1 : Sum  Inputs=++|  InputSameDT=on  SaturateOnIntegerOverflow=on  OutDataTypeStr=Inherit: Same as first input
  Out : Outport  PortDimensions=1
  wires:
  Gain/1 -> Rate Limiter/1  "Ydot"
  Sum/1 -> Gain/1  "Error"
  Integrator/1 -> Sum/1, Out/1  "Y"
  Rate Limiter/1 -> Integrator/1  "Ydot_lim"
  In/1 -> Sum1/2
  Sum1/1 -> Sum/2, Integrator/2
  Constant/1 -> Sum1/1

== system gtm_design_lpv/GTM_T2/Actuators/Acutator Dynamics (Unbiased)/LeftIBSpoilerServo ==
  In : Inport
  Constant : Constant  Value=Bias
  Gain : Gain  Gain=2*pi*freq  SaturateOnIntegerOverflow=on  OutDataTypeStr=Inherit: Same as input  ParamDataTypeStr=Inherit: Same as input
  Integrator : Integrator  InitialConditionSource=external  LimitOutput=on  UpperSaturationLimit=POS_hi  LowerSaturationLimit=POS_lo  IgnoreLimit=on
  Rate Limiter : Saturate  UpperLimit=RL  LowerLimit=-RL
  Sum : Sum  Inputs=-+|  InputSameDT=on  SaturateOnIntegerOverflow=on  OutDataTypeStr=Inherit: Same as first input
  Sum1 : Sum  Inputs=++|  InputSameDT=on  SaturateOnIntegerOverflow=on  OutDataTypeStr=Inherit: Same as first input
  Out : Outport  PortDimensions=1
  wires:
  Gain/1 -> Rate Limiter/1  "Ydot"
  Sum/1 -> Gain/1  "Error"
  Integrator/1 -> Sum/1, Out/1  "Y"
  Rate Limiter/1 -> Integrator/1  "Ydot_lim"
  In/1 -> Sum1/2
  Sum1/1 -> Sum/2, Integrator/2
  Constant/1 -> Sum1/1

== system gtm_design_lpv/GTM_T2/Actuators/Acutator Dynamics (Unbiased)/LeftOBSpoilerServo ==
  In : Inport
  Constant : Constant  Value=Bias
  Gain : Gain  Gain=2*pi*freq  SaturateOnIntegerOverflow=on  OutDataTypeStr=Inherit: Same as input  ParamDataTypeStr=Inherit: Same as input
  Integrator : Integrator  InitialConditionSource=external  LimitOutput=on  UpperSaturationLimit=POS_hi  LowerSaturationLimit=POS_lo  IgnoreLimit=on
  Rate Limiter : Saturate  UpperLimit=RL  LowerLimit=-RL
  Sum : Sum  Inputs=-+|  InputSameDT=on  SaturateOnIntegerOverflow=on  OutDataTypeStr=Inherit: Same as first input
  Sum1 : Sum  Inputs=++|  InputSameDT=on  SaturateOnIntegerOverflow=on  OutDataTypeStr=Inherit: Same as first input
  Out : Outport  PortDimensions=1
  wires:
  Gain/1 -> Rate Limiter/1  "Ydot"
  Sum/1 -> Gain/1  "Error"
  Integrator/1 -> Sum/1, Out/1  "Y"
  Rate Limiter/1 -> Integrator/1  "Ydot_lim"
  In/1 -> Sum1/2
  Sum1/1 -> Sum/2, Integrator/2
  Constant/1 -> Sum1/1

== system gtm_design_lpv/GTM_T2/Actuators/Acutator Dynamics (Unbiased)/RightAileronServo ==
  In : Inport
  Constant : Constant  Value=Bias
  Gain : Gain  Gain=2*pi*freq  SaturateOnIntegerOverflow=on  OutDataTypeStr=Inherit: Same as input  ParamDataTypeStr=Inherit: Same as input
  Integrator : Integrator  InitialConditionSource=external  LimitOutput=on  UpperSaturationLimit=POS_hi  LowerSaturationLimit=POS_lo  IgnoreLimit=on
  Rate Limiter : Saturate  UpperLimit=RL  LowerLimit=-RL
  Sum : Sum  Inputs=-+|  InputSameDT=on  SaturateOnIntegerOverflow=on  OutDataTypeStr=Inherit: Same as first input
  Sum1 : Sum  Inputs=++|  InputSameDT=on  SaturateOnIntegerOverflow=on  OutDataTypeStr=Inherit: Same as first input
  Out : Outport  PortDimensions=1
  wires:
  Gain/1 -> Rate Limiter/1  "Ydot"
  Sum/1 -> Gain/1  "Error"
  Integrator/1 -> Sum/1, Out/1  "Y"
  Rate Limiter/1 -> Integrator/1  "Ydot_lim"
  In/1 -> Sum1/2
  Sum1/1 -> Sum/2, Integrator/2
  Constant/1 -> Sum1/1

== system gtm_design_lpv/GTM_T2/Actuators/Acutator Dynamics (Unbiased)/RightIBSpoilerServo ==
  In : Inport
  Constant : Constant  Value=Bias
  Gain : Gain  Gain=2*pi*freq  SaturateOnIntegerOverflow=on  OutDataTypeStr=Inherit: Same as input  ParamDataTypeStr=Inherit: Same as input
  Integrator : Integrator  InitialConditionSource=external  LimitOutput=on  UpperSaturationLimit=POS_hi  LowerSaturationLimit=POS_lo  IgnoreLimit=on
  Rate Limiter : Saturate  UpperLimit=RL  LowerLimit=-RL
  Sum : Sum  Inputs=-+|  InputSameDT=on  SaturateOnIntegerOverflow=on  OutDataTypeStr=Inherit: Same as first input
  Sum1 : Sum  Inputs=++|  InputSameDT=on  SaturateOnIntegerOverflow=on  OutDataTypeStr=Inherit: Same as first input
  Out : Outport  PortDimensions=1
  wires:
  Gain/1 -> Rate Limiter/1  "Ydot"
  Sum/1 -> Gain/1  "Error"
  Integrator/1 -> Sum/1, Out/1  "Y"
  Rate Limiter/1 -> Integrator/1  "Ydot_lim"
  In/1 -> Sum1/2
  Sum1/1 -> Sum/2, Integrator/2
  Constant/1 -> Sum1/1

== system gtm_design_lpv/GTM_T2/Actuators/Acutator Dynamics (Unbiased)/RightOBSpoilerServo ==
  In : Inport
  Constant : Constant  Value=Bias
  Gain : Gain  Gain=2*pi*freq  SaturateOnIntegerOverflow=on  OutDataTypeStr=Inherit: Same as input  ParamDataTypeStr=Inherit: Same as input
  Integrator : Integrator  InitialConditionSource=external  LimitOutput=on  UpperSaturationLimit=POS_hi  LowerSaturationLimit=POS_lo  IgnoreLimit=on
  Rate Limiter : Saturate  UpperLimit=RL  LowerLimit=-RL
  Sum : Sum  Inputs=-+|  InputSameDT=on  SaturateOnIntegerOverflow=on  OutDataTypeStr=Inherit: Same as first input
  Sum1 : Sum  Inputs=++|  InputSameDT=on  SaturateOnIntegerOverflow=on  OutDataTypeStr=Inherit: Same as first input
  Out : Outport  PortDimensions=1
  wires:
  Gain/1 -> Rate Limiter/1  "Ydot"
  Sum/1 -> Gain/1  "Error"
  Integrator/1 -> Sum/1, Out/1  "Y"
  Rate Limiter/1 -> Integrator/1  "Ydot_lim"
  In/1 -> Sum1/2
  Sum1/1 -> Sum/2, Integrator/2
  Constant/1 -> Sum1/1

== system gtm_design_lpv/GTM_T2/Actuators/Acutator Dynamics (Unbiased)/RudderLServo ==
  In : Inport
  Constant : Constant  Value=Bias
  Gain : Gain  Gain=2*pi*freq  SaturateOnIntegerOverflow=on  OutDataTypeStr=Inherit: Same as input  ParamDataTypeStr=Inherit: Same as input
  Integrator : Integrator  InitialConditionSource=external  LimitOutput=on  UpperSaturationLimit=POS_hi  LowerSaturationLimit=POS_lo  IgnoreLimit=on
  Rate Limiter : Saturate  UpperLimit=RL  LowerLimit=-RL
  Sum : Sum  Inputs=-+|  InputSameDT=on  SaturateOnIntegerOverflow=on  OutDataTypeStr=Inherit: Same as first input
  Sum1 : Sum  Inputs=++|  InputSameDT=on  SaturateOnIntegerOverflow=on  OutDataTypeStr=Inherit: Same as first input
  Out : Outport  PortDimensions=1
  wires:
  Gain/1 -> Rate Limiter/1  "Ydot"
  Sum/1 -> Gain/1  "Error"
  Integrator/1 -> Sum/1, Out/1  "Y"
  Rate Limiter/1 -> Integrator/1  "Ydot_lim"
  In/1 -> Sum1/2
  Sum1/1 -> Sum/2, Integrator/2
  Constant/1 -> Sum1/1

== system gtm_design_lpv/GTM_T2/Actuators/Acutator Dynamics (Unbiased)/RudderUServo ==
  In : Inport
  Constant : Constant  Value=Bias
  Gain : Gain  Gain=2*pi*freq  SaturateOnIntegerOverflow=on  OutDataTypeStr=Inherit: Same as input  ParamDataTypeStr=Inherit: Same as input
  Integrator : Integrator  InitialConditionSource=external  LimitOutput=on  UpperSaturationLimit=POS_hi  LowerSaturationLimit=POS_lo  IgnoreLimit=on
  Rate Limiter : Saturate  UpperLimit=RL  LowerLimit=-RL
  Sum : Sum  Inputs=-+|  InputSameDT=on  SaturateOnIntegerOverflow=on  OutDataTypeStr=Inherit: Same as first input
  Sum1 : Sum  Inputs=++|  InputSameDT=on  SaturateOnIntegerOverflow=on  OutDataTypeStr=Inherit: Same as first input
  Out : Outport  PortDimensions=1
  wires:
  Gain/1 -> Rate Limiter/1  "Ydot"
  Sum/1 -> Gain/1  "Error"
  Integrator/1 -> Sum/1, Out/1  "Y"
  Rate Limiter/1 -> Integrator/1  "Ydot_lim"
  In/1 -> Sum1/2
  Sum1/1 -> Sum/2, Integrator/2
  Constant/1 -> Sum1/1
